simulink model "WaveStar"  (R2018b)
settings: Solver=ode4  StartTime=0  StopTime=141.2  FixedStep=0.001  MaxStep=0.001  RelTol=1e-3  EnableMultiTasking=on
values from neighbouring files (symbols this model uses):
  cc = 10.0    (= 10)    [controller_init.m]
  kc = 0    [controller_init.m]
  L_AB = 0.412    [controller_init.m]
  L_AC = 0.2    [controller_init.m]
  mc = 0    [controller_init.m]
  McSat = inf    [controller_init.m]
  simu = simulationClass()    [wecSimInputFile.m]
  waves = waveClass('irregular')    [wecSimInputFile.m]
  xPcTs = 0.001    [controller_init.m]
undefined symbols (not defined in the file or in its folder): body, constraint, HPfreq, LPfreq, pto, X, Y, Z
libraries: nesl_utility x72, sm_lib x38, WECSim_Lib x7, simulink x2, vrlib x1
(part 2 of 4)

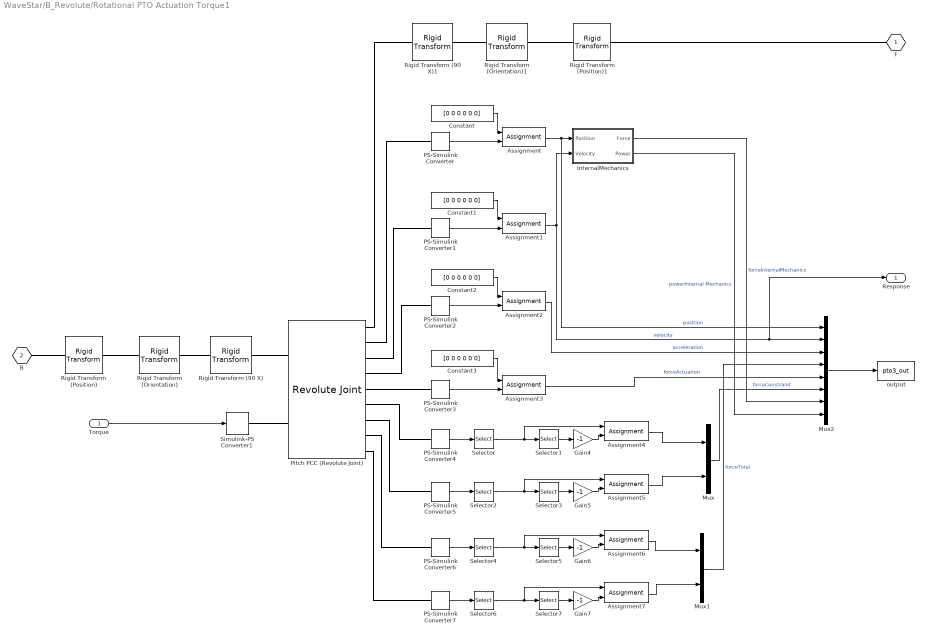
== system WaveStar/B_Revolute/Rotational PTO Actuation Torque1 ==
  Torque : Inport
  "Assignment " : Assignment  IndexOptions=Index vector (dialog)  Indices=5  OutputSizes=1
  Assignment1 : Assignment  IndexOptions=Index vector (dialog)  Indices=5  OutputSizes=1
  Assignment2 : Assignment  IndexOptions=Index vector (dialog)  Indices=5  OutputSizes=1
  Assignment3 : Assignment  IndexOptions=Index vector (dialog)  Indices=5  OutputSizes=1
  Assignment{4..7} (4 alike) : Assignment  DiagnosticForDimensions=Warning  IndexOptions=Index vector (dialog)  Indices=3  OutputSizes=1
  Constant{,1..3} (4 alike) : Constant  Value=[0 0 0 0 0 0]
  Gain{4..7} (4 alike) : Gain  Gain=-1
  InternalMechanics : Subsystem
  Mux : Mux  Inputs=2
  Mux1 : Mux  Inputs=2
  Mux2 : Mux  Inputs=8
  PS-Simulink Converter{,1..7} (8 alike) : nesl_utility/PS-Simulink Converter  PhysicalDomain=network_engine_domain  SubClassName=ps_output  LeftPortType=input  RightPortType=output  PseudoPeriodic=off  Frequencies=[]  Unit=1  AffineConversion=off
  Pitch PCC (Revolute Joint) : sm_lib/Joints/Revolute Joint  SenseConstraintForce=on  SenseConstraintForceX=off  SenseConstraintForceY=off  SenseConstraintForceZ=off  SenseConstraintTorque=on  SenseConstraintTorqueX=off  SenseConstraintTorqueY=off  SenseConstraintTorqueZ=off  SenseTotalForce=on  SenseTotalForceX=off  SenseTotalForceY=off  SenseTotalForceZ=off  SenseTotalTorque=on  SenseTotalTorqueX=off  SenseTotalTorqueY=off  SenseTotalTorqueZ=off  CompositeWrenchDir=BaseOnFollower  CompositeWrenchFrame=BaseFrame  EquilibriumPosition=0  EquilibriumPositionUnits=deg  SpringStiffness=pto.k  SpringStiffnessUnits=N*m/rad  DampingCoefficient=pto.c  DampingCoefficientUnits=N*m/(rad/s)  TorqueActuationMode=InputTorque  MotionActuationMode=ComputedMotion  SensePosition=on  SenseVelocity=on  SenseAcceleration=on  SenseTorqueForce=on  PositionTargetSpecify=off  PositionTargetPriority=High  PositionTargetValue=0  PositionTargetValueUnits=deg  VelocityTargetSpecify=off  VelocityTargetPriority=High  VelocityTargetValue=0  VelocityTargetValueUnits=deg/s
  Rigid Transform (Position) : sm_lib/Frames and Transforms/Rigid Transform  TranslationMethod=Cartesian  TranslationStandardOffset=0  TranslationLengthUnit=m  TranslationStandardAxis=+Z  TranslationCartesianOffset=pto.initDisp.initLinDisp + pto.loc  TranslationROffset=0  TranslationROffsetUnits=m  TranslationZOffset=0  TranslationZOffsetUnits=m  TranslationThetaOffset=0  TranslationThetaOffsetUnits=deg  RotationMethod=None  RotationAngleUnits=rad  RotationStandardAxis=+Y  RotationAngle=0  RotationArbitraryAxis=[0 1 0]  FollAlignAxisA=+X  BaseAlignAxisA=+Y  FollAlignAxisB=+Y  BaseAlignAxisB=+Z  RotationSequenceAxes=FollowerAxes  RotationSequence=XYX  RotationSequenceAngles=[0 0 0]  RotationSequenceAnglesUnits=deg  RotationMatrix=[1 0 0; 0 1 0; 0 0 1]
  Rigid Transform (Position)1 : sm_lib/Frames and Transforms/Rigid Transform  TranslationMethod=Cartesian  TranslationStandardOffset=0  TranslationLengthUnit=m  TranslationStandardAxis=+Z  TranslationCartesianOffset=pto.initDisp.initLinDisp + pto.loc  TranslationROffset=0  TranslationROffsetUnits=m  TranslationZOffset=0  TranslationZOffsetUnits=m  TranslationThetaOffset=0  TranslationThetaOffsetUnits=deg  RotationMethod=None  RotationAngleUnits=rad  RotationStandardAxis=+Y  RotationAngle=0  RotationArbitraryAxis=[0 1 0]  FollAlignAxisA=+X  BaseAlignAxisA=+Y  FollAlignAxisB=+Y  BaseAlignAxisB=+Z  RotationSequenceAxes=FollowerAxes  RotationSequence=XYX  RotationSequenceAngles=[0 0 0]  RotationSequenceAnglesUnits=deg  RotationMatrix=[1 0 0; 0 1 0; 0 0 1]
  Rigid Transform (90 X) : sm_lib/Frames and Transforms/Rigid Transform  TranslationMethod=None  TranslationStandardOffset=0  TranslationLengthUnit=m  TranslationStandardAxis=+Z  TranslationCartesianOffset=0  TranslationROffset=0  TranslationROffsetUnits=m  TranslationZOffset=0  TranslationZOffsetUnits=m  TranslationThetaOffset=0  TranslationThetaOffsetUnits=deg  RotationMethod=StandardAxis  RotationAngleUnits=deg  RotationStandardAxis=+X  RotationAngle=-90  RotationArbitraryAxis=[0 1 0]  FollAlignAxisA=+X  BaseAlignAxisA=+Y  FollAlignAxisB=+Y  BaseAlignAxisB=+Z  RotationSequenceAxes=FollowerAxes  RotationSequence=XYX  RotationSequenceAngles=[0 0 0]  RotationSequenceAnglesUnits=deg  RotationMatrix=[1 0 0; 0 1 0; 0 0 1]
  Rigid Transform (90 X)1 : sm_lib/Frames and Transforms/Rigid Transform  TranslationMethod=None  TranslationStandardOffset=0  TranslationLengthUnit=m  TranslationStandardAxis=+Z  TranslationCartesianOffset=0  TranslationROffset=0  TranslationROffsetUnits=m  TranslationZOffset=0  TranslationZOffsetUnits=m  TranslationThetaOffset=0  TranslationThetaOffsetUnits=deg  RotationMethod=StandardAxis  RotationAngleUnits=deg  RotationStandardAxis=+X  RotationAngle=-90  RotationArbitraryAxis=[0 1 0]  FollAlignAxisA=+X  BaseAlignAxisA=+Y  FollAlignAxisB=+Y  BaseAlignAxisB=+Z  RotationSequenceAxes=FollowerAxes  RotationSequence=XYX  RotationSequenceAngles=[0 0 0]  RotationSequenceAnglesUnits=deg  RotationMatrix=[1 0 0; 0 1 0; 0 0 1]
  Rigid Transform (Orientation) : sm_lib/Frames and Transforms/Rigid Transform  TranslationMethod=None  TranslationStandardOffset=0  TranslationLengthUnit=m  TranslationStandardAxis=+Z  TranslationCartesianOffset=0  TranslationROffset=0  TranslationROffsetUnits=m  TranslationZOffset=0  TranslationZOffsetUnits=m  TranslationThetaOffset=0  TranslationThetaOffsetUnits=deg  RotationMethod=RotationMatrix  RotationAngleUnits=rad  RotationStandardAxis=+Y  RotationAngle=0  RotationArbitraryAxis=[0 1 0]  FollAlignAxisA=+X  BaseAlignAxisA=+Y  FollAlignAxisB=+Y  BaseAlignAxisB=+Z  RotationSequenceAxes=FollowerAxes  RotationSequence=XYX  RotationSequenceAngles=[0 0 0]  RotationSequenceAnglesUnits=deg  RotationMatrix=pto.orientation.rotationMatrix
  Rigid Transform (Orientation)1 : sm_lib/Frames and Transforms/Rigid Transform  TranslationMethod=None  TranslationStandardOffset=0  TranslationLengthUnit=m  TranslationStandardAxis=+Z  TranslationCartesianOffset=0  TranslationROffset=0  TranslationROffsetUnits=m  TranslationZOffset=0  TranslationZOffsetUnits=m  TranslationThetaOffset=0  TranslationThetaOffsetUnits=deg  RotationMethod=RotationMatrix  RotationAngleUnits=rad  RotationStandardAxis=+Y  RotationAngle=0  RotationArbitraryAxis=[0 1 0]  FollAlignAxisA=+X  BaseAlignAxisA=+Y  FollAlignAxisB=+Y  BaseAlignAxisB=+Z  RotationSequenceAxes=FollowerAxes  RotationSequence=XYX  RotationSequenceAngles=[0 0 0]  RotationSequenceAnglesUnits=deg  RotationMatrix=pto.orientation.rotationMatrix
  Selector{,2,4,6} (4 alike) : Selector  InputPortWidth=3  IndexOptions=Index vector (dialog)  Indices=[1 3 2]  OutputSizes=1
  Selector{1,3,5,7} (4 alike) : Selector  InputPortWidth=3  IndexOptions=Index vector (dialog)  Indices=[3]  OutputSizes=1
  Simulink-PS Converter1 : nesl_utility/Simulink-PS Converter  PhysicalDomain=network_engine_domain  SubClassName=ps_input  LeftPortType=input  RightPortType=output  PseudoPeriodic=off  Frequencies=[]  NoiseDistribution=none  NoiseParameters=[]  Unit=1  AffineConversion=off  FilteringAndDerivatives=zero  SimscapeFilterOrder=1  InputFilterTimeConstant=0.001  UdotUserProvided=1
  output : ToWorkspace  VariableName=pto3_out  SaveFormat=Structure With Time  SampleTime=-1
      settings: Decimation=round(simu.dtOut/simu.dt,0)
  F : PMIOPort  Side=Right
  B : PMIOPort  Port=2  Side=Left
  Response : Outport
  wires:
  Torque/1 -> Simulink-PS Converter1/1
  "Assignment "/1 -> Mux2/1, InternalMechanics/1(Position)  "position"
  Assignment1/1 -> Response/1, Mux2/2, InternalMechanics/2(Velocity)  "velocity"
  Assignment2/1 -> Mux2/3  "acceleration"
  Selector2/1 -> Assignment5/1, Selector3/1
  Selector3/1 -> Gain5/1
  Gain5/1 -> Assignment5/2
  Selector/1 -> Assignment4/1, Selector1/1
  Selector1/1 -> Gain4/1
  Gain4/1 -> Assignment4/2
  Assignment5/1 -> Mux/2
  Assignment4/1 -> Mux/1
  Mux/1 -> Mux2/6  "forceConstraint"
  PS-Simulink Converter5/1 -> Selector2/1
  PS-Simulink Converter4/1 -> Selector/1
  Mux2/1 -> output/1
  Mux1/1 -> Mux2/4  "forceTotal"
  Selector6/1 -> Selector7/1, Assignment7/1
  Selector7/1 -> Gain7/1
  Gain7/1 -> Assignment7/2
  Selector4/1 -> Selector5/1, Assignment6/1
  Selector5/1 -> Gain6/1
  Gain6/1 -> Assignment6/2
  PS-Simulink Converter6/1 -> Selector4/1
  PS-Simulink Converter7/1 -> Selector6/1
  Assignment7/1 -> Mux1/2
  Assignment6/1 -> Mux1/1
  Constant/1 -> "Assignment "/1
  PS-Simulink Converter/1 -> "Assignment "/2
  Constant1/1 -> Assignment1/1
  PS-Simulink Converter1/1 -> Assignment1/2
  Constant2/1 -> Assignment2/1
  PS-Simulink Converter2/1 -> Assignment2/2
  Constant3/1 -> Assignment3/1
  PS-Simulink Converter3/1 -> Assignment3/2
  Assignment3/1 -> Mux2/5  "forceActuation"
  InternalMechanics/1(Force) -> Mux2/7  "forceInternalMechanics"
  InternalMechanics/2(Power) -> Mux2/8  "powerInternal Mechanics"
  connections:
  Rigid Transform (Position)1/LConn1 -- F/RConn1
  Rigid Transform (Position)/RConn1 -- Rigid Transform (Orientation)/LConn1
  Rigid Transform (Orientation)/RConn1 -- Rigid Transform (90 X)/LConn1
  Rigid Transform (Orientation)1/RConn1 -- Rigid Transform (90 X)1/LConn1
  Rigid Transform (Position)1/RConn1 -- Rigid Transform (Orientation)1/LConn1
  Rigid Transform (90 X)/RConn1 -- Pitch PCC (Revolute Joint)/LConn1
  Pitch PCC (Revolute Joint)/LConn2 -- Simulink-PS Converter1/RConn1
  Rigid Transform (Position)/LConn1 -- B/RConn1
  PS-Simulink Converter7/LConn1 -- Pitch PCC (Revolute Joint)/RConn9
  PS-Simulink Converter6/LConn1 -- Pitch PCC (Revolute Joint)/RConn8
  PS-Simulink Converter5/LConn1 -- Pitch PCC (Revolute Joint)/RConn7
  PS-Simulink Converter4/LConn1 -- Pitch PCC (Revolute Joint)/RConn6
  Pitch PCC (Revolute Joint)/RConn2 -- PS-Simulink Converter/LConn1
  Pitch PCC (Revolute Joint)/RConn3 -- PS-Simulink Converter1/LConn1
  PS-Simulink Converter2/LConn1 -- Pitch PCC (Revolute Joint)/RConn4
  PS-Simulink Converter3/LConn1 -- Pitch PCC (Revolute Joint)/RConn5
  Rigid Transform (90 X)1/RConn1 -- Pitch PCC (Revolute Joint)/RConn1

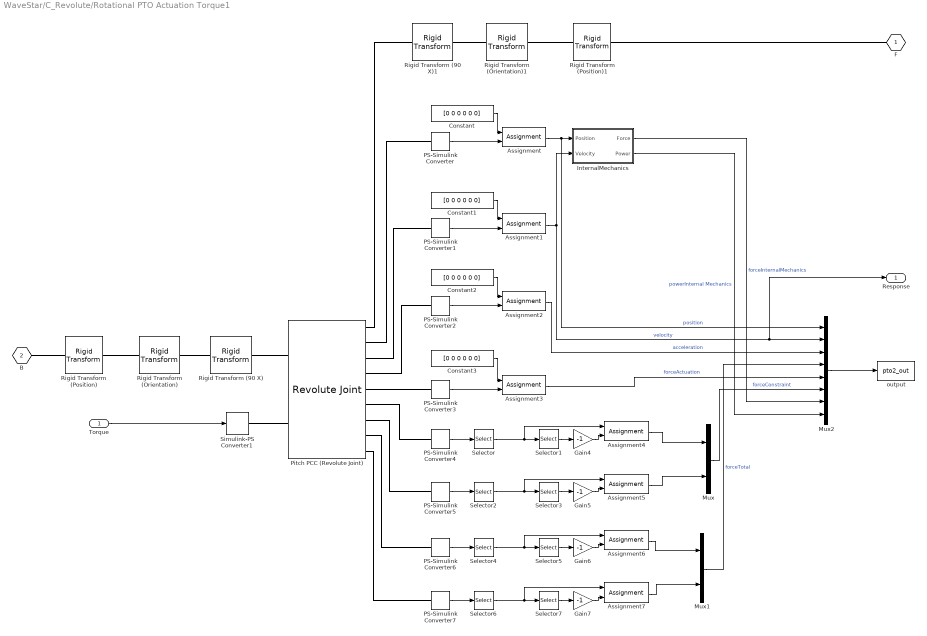
== system WaveStar/C_Revolute/Rotational PTO Actuation Torque1 ==
  Torque : Inport
  "Assignment " : Assignment  IndexOptions=Index vector (dialog)  Indices=5  OutputSizes=1
  Assignment1 : Assignment  IndexOptions=Index vector (dialog)  Indices=5  OutputSizes=1
  Assignment2 : Assignment  IndexOptions=Index vector (dialog)  Indices=5  OutputSizes=1
  Assignment3 : Assignment  IndexOptions=Index vector (dialog)  Indices=5  OutputSizes=1
  Assignment{4..7} (4 alike) : Assignment  DiagnosticForDimensions=Warning  IndexOptions=Index vector (dialog)  Indices=3  OutputSizes=1
  Constant{,1..3} (4 alike) : Constant  Value=[0 0 0 0 0 0]
  Gain{4..7} (4 alike) : Gain  Gain=-1
  InternalMechanics : Subsystem
  Mux : Mux  Inputs=2
  Mux1 : Mux  Inputs=2
  Mux2 : Mux  Inputs=8
  PS-Simulink Converter{,1..7} (8 alike) : nesl_utility/PS-Simulink Converter  PhysicalDomain=network_engine_domain  SubClassName=ps_output  LeftPortType=input  RightPortType=output  PseudoPeriodic=off  Frequencies=[]  Unit=1  AffineConversion=off
  Pitch PCC (Revolute Joint) : sm_lib/Joints/Revolute Joint  SenseConstraintForce=on  SenseConstraintForceX=off  SenseConstraintForceY=off  SenseConstraintForceZ=off  SenseConstraintTorque=on  SenseConstraintTorqueX=off  SenseConstraintTorqueY=off  SenseConstraintTorqueZ=off  SenseTotalForce=on  SenseTotalForceX=off  SenseTotalForceY=off  SenseTotalForceZ=off  SenseTotalTorque=on  SenseTotalTorqueX=off  SenseTotalTorqueY=off  SenseTotalTorqueZ=off  CompositeWrenchDir=BaseOnFollower  CompositeWrenchFrame=BaseFrame  EquilibriumPosition=0  EquilibriumPositionUnits=deg  SpringStiffness=pto.k  SpringStiffnessUnits=N*m/rad  DampingCoefficient=pto.c  DampingCoefficientUnits=N*m/(rad/s)  TorqueActuationMode=InputTorque  MotionActuationMode=ComputedMotion  SensePosition=on  SenseVelocity=on  SenseAcceleration=on  SenseTorqueForce=on  PositionTargetSpecify=off  PositionTargetPriority=High  PositionTargetValue=0  PositionTargetValueUnits=deg  VelocityTargetSpecify=off  VelocityTargetPriority=High  VelocityTargetValue=0  VelocityTargetValueUnits=deg/s
  Rigid Transform (Position) : sm_lib/Frames and Transforms/Rigid Transform  TranslationMethod=Cartesian  TranslationStandardOffset=0  TranslationLengthUnit=m  TranslationStandardAxis=+Z  TranslationCartesianOffset=pto.initDisp.initLinDisp + pto.loc  TranslationROffset=0  TranslationROffsetUnits=m  TranslationZOffset=0  TranslationZOffsetUnits=m  TranslationThetaOffset=0  TranslationThetaOffsetUnits=deg  RotationMethod=None  RotationAngleUnits=rad  RotationStandardAxis=+Y  RotationAngle=0  RotationArbitraryAxis=[0 1 0]  FollAlignAxisA=+X  BaseAlignAxisA=+Y  FollAlignAxisB=+Y  BaseAlignAxisB=+Z  RotationSequenceAxes=FollowerAxes  RotationSequence=XYX  RotationSequenceAngles=[0 0 0]  RotationSequenceAnglesUnits=deg  RotationMatrix=[1 0 0; 0 1 0; 0 0 1]
  Rigid Transform (Position)1 : sm_lib/Frames and Transforms/Rigid Transform  TranslationMethod=Cartesian  TranslationStandardOffset=0  TranslationLengthUnit=m  TranslationStandardAxis=+Z  TranslationCartesianOffset=pto.initDisp.initLinDisp + pto.loc  TranslationROffset=0  TranslationROffsetUnits=m  TranslationZOffset=0  TranslationZOffsetUnits=m  TranslationThetaOffset=0  TranslationThetaOffsetUnits=deg  RotationMethod=None  RotationAngleUnits=rad  RotationStandardAxis=+Y  RotationAngle=0  RotationArbitraryAxis=[0 1 0]  FollAlignAxisA=+X  BaseAlignAxisA=+Y  FollAlignAxisB=+Y  BaseAlignAxisB=+Z  RotationSequenceAxes=FollowerAxes  RotationSequence=XYX  RotationSequenceAngles=[0 0 0]  RotationSequenceAnglesUnits=deg  RotationMatrix=[1 0 0; 0 1 0; 0 0 1]
  Rigid Transform (90 X) : sm_lib/Frames and Transforms/Rigid Transform  TranslationMethod=None  TranslationStandardOffset=0  TranslationLengthUnit=m  TranslationStandardAxis=+Z  TranslationCartesianOffset=0  TranslationROffset=0  TranslationROffsetUnits=m  TranslationZOffset=0  TranslationZOffsetUnits=m  TranslationThetaOffset=0  TranslationThetaOffsetUnits=deg  RotationMethod=StandardAxis  RotationAngleUnits=deg  RotationStandardAxis=+X  RotationAngle=-90  RotationArbitraryAxis=[0 1 0]  FollAlignAxisA=+X  BaseAlignAxisA=+Y  FollAlignAxisB=+Y  BaseAlignAxisB=+Z  RotationSequenceAxes=FollowerAxes  RotationSequence=XYX  RotationSequenceAngles=[0 0 0]  RotationSequenceAnglesUnits=deg  RotationMatrix=[1 0 0; 0 1 0; 0 0 1]
  Rigid Transform (90 X)1 : sm_lib/Frames and Transforms/Rigid Transform  TranslationMethod=None  TranslationStandardOffset=0  TranslationLengthUnit=m  TranslationStandardAxis=+Z  TranslationCartesianOffset=0  TranslationROffset=0  TranslationROffsetUnits=m  TranslationZOffset=0  TranslationZOffsetUnits=m  TranslationThetaOffset=0  TranslationThetaOffsetUnits=deg  RotationMethod=StandardAxis  RotationAngleUnits=deg  RotationStandardAxis=+X  RotationAngle=-90  RotationArbitraryAxis=[0 1 0]  FollAlignAxisA=+X  BaseAlignAxisA=+Y  FollAlignAxisB=+Y  BaseAlignAxisB=+Z  RotationSequenceAxes=FollowerAxes  RotationSequence=XYX  RotationSequenceAngles=[0 0 0]  RotationSequenceAnglesUnits=deg  RotationMatrix=[1 0 0; 0 1 0; 0 0 1]
  Rigid Transform (Orientation) : sm_lib/Frames and Transforms/Rigid Transform  TranslationMethod=None  TranslationStandardOffset=0  TranslationLengthUnit=m  TranslationStandardAxis=+Z  TranslationCartesianOffset=0  TranslationROffset=0  TranslationROffsetUnits=m  TranslationZOffset=0  TranslationZOffsetUnits=m  TranslationThetaOffset=0  TranslationThetaOffsetUnits=deg  RotationMethod=RotationMatrix  RotationAngleUnits=rad  RotationStandardAxis=+Y  RotationAngle=0  RotationArbitraryAxis=[0 1 0]  FollAlignAxisA=+X  BaseAlignAxisA=+Y  FollAlignAxisB=+Y  BaseAlignAxisB=+Z  RotationSequenceAxes=FollowerAxes  RotationSequence=XYX  RotationSequenceAngles=[0 0 0]  RotationSequenceAnglesUnits=deg  RotationMatrix=pto.orientation.rotationMatrix
  Rigid Transform (Orientation)1 : sm_lib/Frames and Transforms/Rigid Transform  TranslationMethod=None  TranslationStandardOffset=0  TranslationLengthUnit=m  TranslationStandardAxis=+Z  TranslationCartesianOffset=0  TranslationROffset=0  TranslationROffsetUnits=m  TranslationZOffset=0  TranslationZOffsetUnits=m  TranslationThetaOffset=0  TranslationThetaOffsetUnits=deg  RotationMethod=RotationMatrix  RotationAngleUnits=rad  RotationStandardAxis=+Y  RotationAngle=0  RotationArbitraryAxis=[0 1 0]  FollAlignAxisA=+X  BaseAlignAxisA=+Y  FollAlignAxisB=+Y  BaseAlignAxisB=+Z  RotationSequenceAxes=FollowerAxes  RotationSequence=XYX  RotationSequenceAngles=[0 0 0]  RotationSequenceAnglesUnits=deg  RotationMatrix=pto.orientation.rotationMatrix
  Selector{,2,4,6} (4 alike) : Selector  InputPortWidth=3  IndexOptions=Index vector (dialog)  Indices=[1 3 2]  OutputSizes=1
  Selector{1,3,5,7} (4 alike) : Selector  InputPortWidth=3  IndexOptions=Index vector (dialog)  Indices=[3]  OutputSizes=1
  Simulink-PS Converter1 : nesl_utility/Simulink-PS Converter  PhysicalDomain=network_engine_domain  SubClassName=ps_input  LeftPortType=input  RightPortType=output  PseudoPeriodic=off  Frequencies=[]  NoiseDistribution=none  NoiseParameters=[]  Unit=1  AffineConversion=off  FilteringAndDerivatives=zero  SimscapeFilterOrder=1  InputFilterTimeConstant=0.001  UdotUserProvided=1
  output : ToWorkspace  VariableName=pto2_out  SaveFormat=Structure With Time  SampleTime=-1
      settings: Decimation=round(simu.dtOut/simu.dt,0)
  F : PMIOPort  Side=Right
  B : PMIOPort  Port=2  Side=Left
  Response : Outport
  wires:
  Torque/1 -> Simulink-PS Converter1/1
  "Assignment "/1 -> Mux2/1, InternalMechanics/1(Position)  "position"
  Assignment1/1 -> Response/1, Mux2/2, InternalMechanics/2(Velocity)  "velocity"
  Assignment2/1 -> Mux2/3  "acceleration"
  Selector2/1 -> Assignment5/1, Selector3/1
  Selector3/1 -> Gain5/1
  Gain5/1 -> Assignment5/2
  Selector/1 -> Assignment4/1, Selector1/1
  Selector1/1 -> Gain4/1
  Gain4/1 -> Assignment4/2
  Assignment5/1 -> Mux/2
  Assignment4/1 -> Mux/1
  Mux/1 -> Mux2/6  "forceConstraint"
  PS-Simulink Converter5/1 -> Selector2/1
  PS-Simulink Converter4/1 -> Selector/1
  Mux2/1 -> output/1
  Mux1/1 -> Mux2/4  "forceTotal"
  Selector6/1 -> Selector7/1, Assignment7/1
  Selector7/1 -> Gain7/1
  Gain7/1 -> Assignment7/2
  Selector4/1 -> Selector5/1, Assignment6/1
  Selector5/1 -> Gain6/1
  Gain6/1 -> Assignment6/2
  PS-Simulink Converter6/1 -> Selector4/1
  PS-Simulink Converter7/1 -> Selector6/1
  Assignment7/1 -> Mux1/2
  Assignment6/1 -> Mux1/1
  Constant/1 -> "Assignment "/1
  PS-Simulink Converter/1 -> "Assignment "/2
  Constant1/1 -> Assignment1/1
  PS-Simulink Converter1/1 -> Assignment1/2
  Constant2/1 -> Assignment2/1
  PS-Simulink Converter2/1 -> Assignment2/2
  Constant3/1 -> Assignment3/1
  PS-Simulink Converter3/1 -> Assignment3/2
  Assignment3/1 -> Mux2/5  "forceActuation"
  InternalMechanics/1(Force) -> Mux2/7  "forceInternalMechanics"
  InternalMechanics/2(Power) -> Mux2/8  "powerInternal Mechanics"
  connections:
  Rigid Transform (Position)1/LConn1 -- F/RConn1
  Rigid Transform (Position)/RConn1 -- Rigid Transform (Orientation)/LConn1
  Rigid Transform (Orientation)/RConn1 -- Rigid Transform (90 X)/LConn1
  Rigid Transform (Orientation)1/RConn1 -- Rigid Transform (90 X)1/LConn1
  Rigid Transform (Position)1/RConn1 -- Rigid Transform (Orientation)1/LConn1
  Rigid Transform (90 X)/RConn1 -- Pitch PCC (Revolute Joint)/LConn1
  Pitch PCC (Revolute Joint)/LConn2 -- Simulink-PS Converter1/RConn1
  Rigid Transform (Position)/LConn1 -- B/RConn1
  PS-Simulink Converter7/LConn1 -- Pitch PCC (Revolute Joint)/RConn9
  PS-Simulink Converter6/LConn1 -- Pitch PCC (Revolute Joint)/RConn8
  PS-Simulink Converter5/LConn1 -- Pitch PCC (Revolute Joint)/RConn7
  PS-Simulink Converter4/LConn1 -- Pitch PCC (Revolute Joint)/RConn6
  Pitch PCC (Revolute Joint)/RConn2 -- PS-Simulink Converter/LConn1
  Pitch PCC (Revolute Joint)/RConn3 -- PS-Simulink Converter1/LConn1
  PS-Simulink Converter2/LConn1 -- Pitch PCC (Revolute Joint)/RConn4
  PS-Simulink Converter3/LConn1 -- Pitch PCC (Revolute Joint)/RConn5
  Rigid Transform (90 X)1/RConn1 -- Pitch PCC (Revolute Joint)/RConn1

== system WaveStar/Controller/Linear ==
  wave_gauge_1 : Inport
  wave_gauge_2 : Inport  Port=2
  wave_gauge_3 : Inport  Port=3
  float_accel : Inport  Port=4
  motor_force : Inport  Port=5
  "motor_pos " : Inport  Port=6
  WECCCOMP Controller : Subsystem
  cmd_force : Outport
  wires:
  WECCCOMP Controller/1(cmd_force) -> cmd_force/1
  float_accel/1 -> WECCCOMP Controller/1(float_accel_rot)
  motor_force/1 -> WECCCOMP Controller/2(motor_force)
  "motor_pos "/1 -> WECCCOMP Controller/3("motor_pos ")
  wave_gauge_1/1 -> WECCCOMP Controller/4(wave_gauge_1)
  wave_gauge_2/1 -> WECCCOMP Controller/5(wave_gauge_2)
  wave_gauge_3/1 -> WECCCOMP Controller/6(wave_gauge_3)

== system WaveStar/Controller/Rotary ==
  wave_gauge_1 : Inport
  wave_gauge_2 : Inport  Port=2
  wave_gauge_3 : Inport  Port=3
  float_accel : Inport  Port=4
  motor_force : Inport  Port=5
  "motor_pos " : Inport  Port=6
  MATLAB Function : MATLAB Function  TreatAsAtomicUnit=on
  Ramp : simulink/Sources/Ramp  slope=1  start=0  InitialOutput=0
  Rate Transition1 : RateTransition  OutPortSampleTime=simu.dt
  WECCCOMP Controller : Subsystem
  lin2rot conversion : Subsystem
  rot2lin conversion : Subsystem
  cmd_force : Outport
  wires:
  float_accel/1 -> lin2rot conversion/1(float_accel)
  motor_force/1 -> lin2rot conversion/2(motor_force)
  "motor_pos "/1 -> lin2rot conversion/3("motor_pos ")
  rot2lin conversion/1(cmd_force) -> cmd_force/1
  WECCCOMP Controller/1(cmd_torque_rot) -> rot2lin conversion/1(cmd_torque_rot)
  lin2rot conversion/2(motor_torque_rot) -> WECCCOMP Controller/2(motor_torque_rot)
  lin2rot conversion/1("float_accel_rot ") -> MATLAB Function/4(float_accel)
  lin2rot conversion/3(motor_pos_rot) -> MATLAB Function/6(pos)
  wave_gauge_1/1 -> MATLAB Function/1(ws1)
  lin2rot conversion/4(moment_arm) -> rot2lin conversion/2(moment_arm)
  wave_gauge_2/1 -> MATLAB Function/2(ws2)
  wave_gauge_3/1 -> MATLAB Function/3(ws3)
  MATLAB Function/1(WS1) -> WECCCOMP Controller/4(wave_gauge_1)
  MATLAB Function/2(WS2) -> WECCCOMP Controller/5(wave_gauge_2)
  MATLAB Function/3(WS3) -> WECCCOMP Controller/6(wave_gauge_3)
  MATLAB Function/4(ACC) -> WECCCOMP Controller/1(float_accel_rot)
  MATLAB Function/5(POS) -> WECCCOMP Controller/3("motor_pos_rot ")
  Ramp/1 -> Rate Transition1/1
  Rate Transition1/1 -> MATLAB Function/5(time)

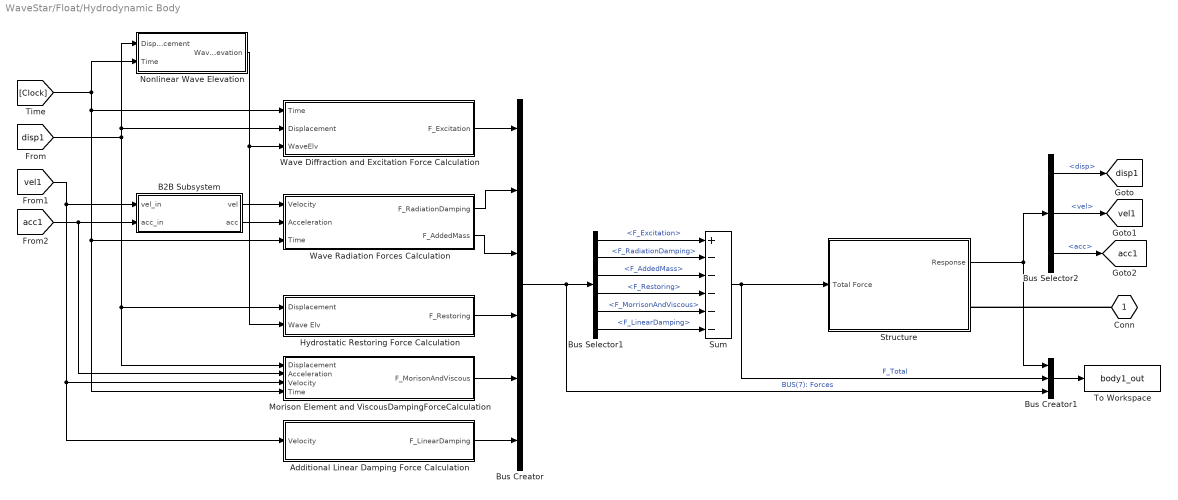
== system WaveStar/Float/Hydrodynamic Body ==
  Additional Linear Damping Force Calculation : Subsystem
  B2B Subsystem : Subsystem  Variant=on
  Bus Creator : BusCreator  Inputs=6
  Bus Creator1 : BusCreator  Inputs=3
  Bus Selector1 : BusSelector  OutputSignals=F_Excitation,F_RadiationDamping,F_AddedMass,F_Restoring,F_MorrisonAndViscous,F_LinearDamping
  Bus Selector2 : BusSelector  OutputSignals=disp,vel,acc
  Hydrostatic Restoring Force Calculation : Subsystem
  Morison Element and ViscousDampingForceCalculation : Subsystem
  Nonlinear Wave Elevation : Subsystem  TreatAsAtomicUnit=on  SystemSampleTime=simu.dtNL
  Structure : Subsystem
  Sum : Sum  Inputs=+-----
  To Workspace : ToWorkspace  VariableName=body1_out  SaveFormat=Structure With Time  SampleTime=-1
      settings: Decimation=round(simu.dtOut/simu.dt,0)
  Wave Diffraction and Excitation Force Calculation : Subsystem
  Wave Radiation Forces Calculation : Subsystem
  Conn : PMIOPort  Side=Right
  tag scope: acc1=global, disp1=global, vel1=global
  wires:
  Additional Linear Damping Force Calculation/1(F_LinearDamping) -> Bus Creator/6
  Bus Creator/1 -> Bus Selector1/1, Bus Creator1/3  "BUS(7): Forces"
  Bus Selector2/1 -> [disp1]  "<disp>"
  Bus Selector2/3 -> [acc1]  "<acc>"
  Bus Selector2/2 -> [vel1]  "<vel>"
  Structure/1(Response) -> Bus Creator1/1, Bus Selector2/1
  Sum/1 -> Bus Creator1/2, Structure/1(Total Force)  "F_Total"
  Bus Creator1/1 -> To Workspace/1
  Bus Selector1/4 -> Sum/4  "<F_Restoring>"
  Bus Selector1/3 -> Sum/3  "<F_AddedMass>"
  Bus Selector1/5 -> Sum/5  "<F_MorrisonAndViscous>"
  Bus Selector1/2 -> Sum/2  "<F_RadiationDamping>"
  Bus Selector1/1 -> Sum/1  "<F_Excitation>"
  Bus Selector1/6 -> Sum/6  "<F_LinearDamping>"
  [acc1] -> B2B Subsystem/2(acc_in), Morison Element and ViscousDampingForceCalculation/2(Acceleration)
  [vel1] -> Morison Element and ViscousDampingForceCalculation/3(Velocity), Additional Linear Damping Force Calculation/1(Velocity), B2B Subsystem/1(vel_in)
  B2B Subsystem/2(acc) -> Wave Radiation Forces Calculation/2(Acceleration)
  B2B Subsystem/1(vel) -> Wave Radiation Forces Calculation/1(Velocity)
  [disp1] -> Hydrostatic Restoring Force Calculation/1(Displacement), Morison Element and ViscousDampingForceCalculation/1(Displacement), Nonlinear Wave Elevation/1(Displacement), Wave Diffraction and Excitation Force Calculation/2(Displacement)
  Nonlinear Wave Elevation/1(Wave Elevation) -> Wave Diffraction and Excitation Force Calculation/3(WaveElv), Hydrostatic Restoring Force Calculation/2(Wave Elv)
  Hydrostatic Restoring Force Calculation/1(F_Restoring) -> Bus Creator/4
  Wave Radiation Forces Calculation/1(F_RadiationDamping) -> Bus Creator/2
  Wave Diffraction and Excitation Force Calculation/1(F_Excitation) -> Bus Creator/1
  Wave Radiation Forces Calculation/2(F_AddedMass) -> Bus Creator/3
  [Clock] -> Nonlinear Wave Elevation/2(Time), Wave Diffraction and Excitation Force Calculation/1(Time), Morison Element and ViscousDampingForceCalculation/4(Time), Wave Radiation Forces Calculation/3(Time)
  Morison Element and ViscousDampingForceCalculation/1(F_MorisonAndViscous) -> Bus Creator/5
  connections:
  Conn/RConn1 -- Structure/RConn1

== system WaveStar/Float/Non-Hydro Body ==
  Bus Creator : BusCreator  Inputs=6
  Bus Creator1 : BusCreator  Inputs=3
  Bus Selector1 : BusSelector  OutputSignals=F_Excitation,F_RadiationDamping,F_AddedMass,F_Restoring,F_MorrisonAndViscous,F_LinearDamping
  Constant{,1..3,5} (5 alike) : Constant  Value=[0 0 0 0 0 0]
  Structure : Subsystem
  Sum : Sum  Inputs=+-----
  To Workspace : ToWorkspace  VariableName=body1_out  SaveFormat=Structure With Time  SampleTime=-1
      settings: Decimation=round(simu.dtOut/simu.dt,0)
  Weight and Buoyancy : Subsystem
  Conn : PMIOPort  Side=Right
  wires:
  Bus Creator/1 -> Bus Creator1/3, Bus Selector1/1  "BUS(7): Forces"
  Structure/1(Response) -> Bus Creator1/1
  Sum/1 -> Bus Creator1/2, Structure/1(Total Force)  "F_Total"
  Bus Creator1/1 -> To Workspace/1
  Bus Selector1/4 -> Sum/4  "<F_Restoring>"
  Bus Selector1/3 -> Sum/3  "<F_AddedMass>"
  Bus Selector1/5 -> Sum/5  "<F_MorrisonAndViscous>"
  Bus Selector1/2 -> Sum/2  "<F_RadiationDamping>"
  Bus Selector1/1 -> Sum/1  "<F_Excitation>"
  Bus Selector1/6 -> Sum/6  "<F_LinearDamping>"
  Constant5/1 -> Bus Creator/6  "F_LinearDamping"
  Constant3/1 -> Bus Creator/5  "F_MorrisonAndViscous"
  Constant2/1 -> Bus Creator/3  "F_AddedMass"
  Constant1/1 -> Bus Creator/2  "F_RadiationDamping"
  Constant/1 -> Bus Creator/1  "F_Excitation"
  Weight and Buoyancy/1(Out1) -> Bus Creator/4  "F_Restoring"
  connections:
  Conn/RConn1 -- Structure/RConn1

== system WaveStar/Linear Motor/InternalMechanics ==
  note: Calculate PTO force and power.
      |
      | F_pto  = k*x + c*v,
      | where F_pto is the force the PTO applies to the body (at the PTO location), x and v are the joint position and velocity.
      |
      | The power extracted is
      | P = c * v^2
  Position : Inport
  Velocity : Inport  Port=2
  Add : Sum  Inputs=--
  Math Function : Math  Operator=square  SaturateOnIntegerOverflow=on
  PCC Damping Coefficient : Constant  Value=pto.c
  PCC Stiffness Coefficient : Constant  Value=pto.k
  Product : Product  Inputs=**
  Product1 : Product  Inputs=**
  Product2 : Product  Inputs=**
  Force : Outport
  Power : Outport  Port=2
  wires:
  PCC Damping Coefficient/1 -> Product2/1, Product1/1
  Product2/1 -> Power/1
  Velocity/1 -> Math Function/1, Product1/2
  PCC Stiffness Coefficient/1 -> Product/2
  Position/1 -> Product/1
  Add/1 -> Force/1
  Math Function/1 -> Product2/2
  Product/1 -> Add/1
  Product1/1 -> Add/2

== system WaveStar/A_Revolute/Rotational PTO Actuation Torque1/InternalMechanics ==
  note: Calculate PTO force and power.
      |
      | F_pto  = k*x + c*v,
      | where F_pto is the force the PTO applies to the body (at the PTO location), x and v are the joint position and velocity.
      |
      | The power extracted is
      | P_pto = F_pto * v
  Position : Inport
  Velocity : Inport  Port=2
  Add : Sum  Inputs=--
  PCC Damping Coefficient : Constant  Value=pto.c
  PCC Stiffness Coefficient : Constant  Value=pto.k
  Product : Product  Inputs=**
  Product1 : Product  Inputs=**
  Product2 : Product  Inputs=**
  Force : Outport
  Power : Outport  Port=2
  wires:
  PCC Damping Coefficient/1 -> Product1/1
  Product2/1 -> Power/1
  PCC Stiffness Coefficient/1 -> Product/2
  Position/1 -> Product/1
  Add/1 -> Force/1, Product2/1
  Velocity/1 -> Product1/2, Product2/2
  Product/1 -> Add/1
  Product1/1 -> Add/2

== system WaveStar/B_Revolute/Rotational PTO Actuation Torque1/InternalMechanics ==
  note: Calculate PTO force and power.
      |
      | F_pto  = k*x + c*v,
      | where F_pto is the force the PTO applies to the body (at the PTO location), x and v are the joint position and velocity.
      |
      | The power extracted is
      | P_pto = F_pto * v
  Position : Inport
  Velocity : Inport  Port=2
  Add : Sum  Inputs=--
  PCC Damping Coefficient : Constant  Value=pto.c
  PCC Stiffness Coefficient : Constant  Value=pto.k
  Product : Product  Inputs=**
  Product1 : Product  Inputs=**
  Product2 : Product  Inputs=**
  Force : Outport
  Power : Outport  Port=2
  wires:
  PCC Damping Coefficient/1 -> Product1/1
  Product2/1 -> Power/1
  PCC Stiffness Coefficient/1 -> Product/2
  Position/1 -> Product/1
  Add/1 -> Force/1, Product2/1
  Velocity/1 -> Product1/2, Product2/2
  Product/1 -> Add/1
  Product1/1 -> Add/2

== system WaveStar/C_Revolute/Rotational PTO Actuation Torque1/InternalMechanics ==
  note: Calculate PTO force and power.
      |
      | F_pto  = k*x + c*v,
      | where F_pto is the force the PTO applies to the body (at the PTO location), x and v are the joint position and velocity.
      |
      | The power extracted is
      | P_pto = F_pto * v
  Position : Inport
  Velocity : Inport  Port=2
  Add : Sum  Inputs=--
  PCC Damping Coefficient : Constant  Value=pto.c
  PCC Stiffness Coefficient : Constant  Value=pto.k
  Product : Product  Inputs=**
  Product1 : Product  Inputs=**
  Product2 : Product  Inputs=**
  Force : Outport
  Power : Outport  Port=2
  wires:
  PCC Damping Coefficient/1 -> Product1/1
  Product2/1 -> Power/1
  PCC Stiffness Coefficient/1 -> Product/2
  Position/1 -> Product/1
  Add/1 -> Force/1, Product2/1
  Velocity/1 -> Product1/2, Product2/2
  Product/1 -> Add/1
  Product1/1 -> Add/2

== system WaveStar/Controller/Linear/WECCCOMP Controller ==
  float_accel_rot : Inport
  motor_force : Inport  Port=2
  "motor_pos " : Inport  Port=3
  wave_gauge_1 : Inport  Port=4
  wave_gauge_2 : Inport  Port=5
  wave_gauge_3 : Inport  Port=6
  Constant : Constant  Value=0
  Terminator{,1..5} (6 alike) : Terminator
  lin2rot conversion : Subsystem
  rot2lin conversion : Subsystem
  cmd_force : Outport
  wires:
  lin2rot conversion/2(moment_arm) -> rot2lin conversion/2(moment_arm)
  wave_gauge_1/1 -> Terminator/1
  "motor_pos "/1 -> lin2rot conversion/2("motor_pos ")
  motor_force/1 -> Terminator2/1
  float_accel_rot/1 -> lin2rot conversion/1(float_accel_rot)
  rot2lin conversion/1(cmd_force) -> cmd_force/1
  Constant/1 -> rot2lin conversion/1(cmd_force_ref)
  lin2rot conversion/1("float_accel ") -> Terminator1/1
  lin2rot conversion/3(motor_vel) -> Terminator4/1
  wave_gauge_2/1 -> Terminator3/1
  wave_gauge_3/1 -> Terminator5/1

== system WaveStar/Controller/Rotary/WECCCOMP Controller ==
  float_accel_rot : Inport
  motor_torque_rot : Inport  Port=2
  "motor_pos_rot " : Inport  Port=3
  wave_gauge_1 : Inport  Port=4
  wave_gauge_2 : Inport  Port=5
  wave_gauge_3 : Inport  Port=6
  Differentiator with break frequency : DiscreteTransferFcn  Numerator=[1 -1]*2*2*pi*HPfreq.vel  Denominator=[(2+2*pi*HPfreq.vel*xPcTs) (2*pi*HPfreq.vel*xPcTs-2)]
  First order LP filter : DiscreteTransferFcn  Numerator=[1 1]*xPcTs*2*pi*LPfreq.vel  Denominator=[(2+xPcTs*2*pi*LPfreq.vel) (xPcTs*2*pi*LPfreq.vel-2)]
  Sum1 : Sum  Inputs=+++
  cc : Gain  Gain=cc
  kc : Gain  Gain=kc
  mc : Gain  Gain=mc
  motor torque terminator : Terminator
  wave gauge 1 terminator : Terminator
  wave gauge 2 terminator : Terminator
  wave gauge 3 terminator : Terminator
  cmd_torque_rot : Outport
  wires:
  cc/1 -> Sum1/2
  kc/1 -> Sum1/3
  "motor_pos_rot "/1 -> Differentiator with break frequency/1, kc/1
  float_accel_rot/1 -> mc/1
  mc/1 -> Sum1/1
  motor_torque_rot/1 -> motor torque terminator/1
  wave_gauge_1/1 -> wave gauge 1 terminator/1
  Differentiator with break frequency/1 -> First order LP filter/1
  First order LP filter/1 -> cc/1
  Sum1/1 -> cmd_torque_rot/1  "Mc"
  wave_gauge_2/1 -> wave gauge 2 terminator/1
  wave_gauge_3/1 -> wave gauge 3 terminator/1

== system WaveStar/Controller/Rotary/lin2rot conversion ==
  float_accel : Inport
  motor_force : Inport  Port=2
  "motor_pos " : Inport  Port=3
  Axial Motor Force : Selector  InputPortWidth=6  IndexOptions=Index vector (dialog)  Indices=[3]  OutputSizes=1
  Axial Position : Selector  InputPortWidth=6  IndexOptions=Index vector (dialog)  Indices=[3]  OutputSizes=1
  Divide => K (m)2 : Product  Inputs=**
  Linear2Angular Conversion : Subsystem
  "float_accel_rot " : Outport
  motor_torque_rot : Outport  Port=2
  motor_pos_rot : Outport  Port=3
  moment_arm : Outport  Port=4
  wires:
  "motor_pos "/1 -> Axial Position/1
  Linear2Angular Conversion/2(moment_arm) -> Divide => K (m)2/1, moment_arm/1
  Axial Position/1 -> Linear2Angular Conversion/1(x_cyl)
  Linear2Angular Conversion/1(Theta) -> motor_pos_rot/1
  float_accel/1 -> "float_accel_rot "/1  "Angular Acceleration"
  motor_force/1 -> Axial Motor Force/1
  Axial Motor Force/1 -> Divide => K (m)2/2
  Divide => K (m)2/1 -> motor_torque_rot/1

== system WaveStar/Controller/Rotary/rot2lin conversion ==
  cmd_torque_rot : Inport
  moment_arm : Inport  Port=2
  Cmd torque to measured torque dynamics : DiscreteTransferFcn  Numerator="[0.96294775   -1.92342278    0.96053421]"  Denominator="[1.00000000   -1.99777700    0.99783206]"
  "Divide " : Product  Inputs=*/
  Gain : Gain  Gain=-1
  Saturation : Saturate  UpperLimit=McSat  LowerLimit=-McSat
  cmd_force : Outport
  wires:
  "Divide "/1 -> cmd_force/1
  moment_arm/1 -> "Divide "/2
  Saturation/1 -> Gain/1  "Mc_sat"
  Gain/1 -> "Divide "/1
  cmd_torque_rot/1 -> Cmd torque to measured torque dynamics/1
  Cmd torque to measured torque dynamics/1 -> Saturation/1

== system WaveStar/Float/Hydrodynamic Body/Additional Linear Damping Force Calculation ==
  Velocity : Inport
  Additional Linear Damping Matrix (diagonal) : Constant  Value=body.hydroForce.linearDamping
  Product1 : Product
  F_LinearDamping : Outport
  wires:
  Velocity/1 -> Product1/2  "v"
  Product1/1 -> F_LinearDamping/1  "F_LinearDamping"
  Additional Linear Damping Matrix (diagonal)/1 -> Product1/1  "C"

== system WaveStar/Float/Hydrodynamic Body/B2B Subsystem ==
  note: 1) Add Subsystem or Model blocks as valid variant choices.
      | 2) You cannot connect blocks at this level. At simulation, connectivity is automatically
      | determined, based on the active variant and port name matching.
  vel_in : Inport
  acc_in : Inport  Port=2
  B2B : Subsystem  VariantControl=sv_B2B
  noB2B : Subsystem  VariantControl=sv_noB2B
  vel : Outport
  acc : Outport  Port=2

== system WaveStar/Float/Hydrodynamic Body/Hydrostatic Restoring Force Calculation ==
  Displacement : Inport
  Wave Elv : Inport  Port=2
  Add : Sum  Inputs=+-
  Center of Gravity : Constant  Value=body.cg
  Constant : Constant  Value=zeros(1,body.dof-3)
  Linear and Nonlinear Restoring Force Variant Subsystem : Subsystem  Variant=on
  Mux : Mux  Inputs=2
  F_Restoring : Outport
  wires:
  Add/1 -> Linear and Nonlinear Restoring Force Variant Subsystem/1(In1)  "x_cg"
  Wave Elv/1 -> Linear and Nonlinear Restoring Force Variant Subsystem/2(In2)
  Constant/1 -> Mux/2
  Center of Gravity/1 -> Mux/1  "cg"
  Mux/1 -> Add/2
  Linear and Nonlinear Restoring Force Variant Subsystem/1(Out1) -> F_Restoring/1  "F_Restoring"
  Displacement/1 -> Add/1  "x"

== system WaveStar/Float/Hydrodynamic Body/Morison Element and ViscousDampingForceCalculation ==
  Displacement : Inport
  Acceleration : Inport  Port=2
  Velocity : Inport  Port=3
  Time : Inport  Port=4
  Abs1 : Abs
  Morison Element Variant Subsystem : Subsystem  Variant=on
  Product : Product
  Product1 : Product  Multiplication=Matrix(*)
  Transport Delay : TransportDelay  DelayTime=10e-8
  "VisSum " : Sum  Inputs=+-
  "Viscous Damping Matrix (diagonal) " : Constant  Value=body.hydroForce.visDrag
  F_MorisonAndViscous : Outport
  wires:
  Morison Element Variant Subsystem/1(morison_force) -> "VisSum "/2
  Velocity/1 -> Abs1/1, Morison Element Variant Subsystem/2(velocity), Product/1
  Transport Delay/1 -> Morison Element Variant Subsystem/3(acceleration)
  Displacement/1 -> Morison Element Variant Subsystem/1(displacement)
  Time/1 -> Morison Element Variant Subsystem/4(time)
  Product/1 -> Product1/2  "v * |v|"
  "Viscous Damping Matrix (diagonal) "/1 -> Product1/1  "0.5 * cd * rho *A"
  Product1/1 -> "VisSum "/1
  Abs1/1 -> Product/2
  Acceleration/1 -> Transport Delay/1
  "VisSum "/1 -> F_MorisonAndViscous/1  "F_MorrisonAndViscous"

== system WaveStar/Float/Hydrodynamic Body/Nonlinear Wave Elevation ==
  Displacement : Inport
  Time : Inport  Port=2
  Add : Sum  Inputs=+-
  Center of Gravity : Constant  Value=body.cg
  Constant : Constant  Value=zeros(1,body.dof-3)
  Linear or Instantaneous Free Surface : Subsystem  Variant=on
  Mux : Mux  Inputs=2
  Wave Elevation : Outport
  wires:
  Time/1 -> Linear or Instantaneous Free Surface/2(In2)
  Constant/1 -> Mux/2
  Center of Gravity/1 -> Mux/1  "cg"
  Mux/1 -> Add/2
  Add/1 -> Linear or Instantaneous Free Surface/1(In1)  "x_cg"
  Linear or Instantaneous Free Surface/1(Out1) -> Wave Elevation/1
  Displacement/1 -> Add/1  "x"

== system WaveStar/Float/Hydrodynamic Body/Structure ==
  Total Force : Inport
  Body Properties : sm_lib/Body Elements/Solid  InertiaType=Custom  Mass=body.mass  MassUnits=kg  CenterOfMass=[0 0 0]  CenterOfMassUnits=m  MomentsOfInertia=body.momOfInertia  MomentsOfInertiaUnits=kg*m^2  ProductsOfInertia=[0 0 0]  ProductsOfInertiaUnits=kg*m^2  BasedOnType=Density  Density=1000  DensityUnits=kg/(m^3)  DoExposeReferenceFrame=on  SerializedFrames=<Frames/>  GraphicType=FromGeometry  MarkerShape=Sphere  MarkerSize=10  MarkerSizeUnits=m  GraphicVisPropType=SimpleVisualProperties  GraphicDiffuseColor=body.viz.color  GraphicSpecularColor=[0.5 0.5 0.5 1.0]  GraphicAmbientColor=[0.15 0.15 0.15 1.0]  GraphicEmissiveColor=[0.0 0.0 0.0 1.0]  GraphicShininess=75  GraphicOpacity=body.viz.opacity  GeometryShape=FromFile  RectangleSize=[1 1]  RectangleSizeUnits=m  BrickDimensions=[1 1 1]  BrickDimensionUnits=m  CylinderRadius=1  CylinderRadiusUnits=m  CylinderLength=1  CylinderLengthUnits=m  SphereRadius=1  SphereRadiusUnits=m  EllipsoidRadii=[1 1 1]  EllipsoidRadiiUnits=m  ExtrusionCrossSection=[1 1; -1 1; -1 -1; 1 -1]  ExtrusionCrossSectionUnits=m  ExtrusionLength=1  ExtrusionLengthUnits=m  PolygonNumSides=3  PolygonOuterRadius=1  PolygonOuterRadiusUnits=m  ExtGeomFileType=STL  ExtGeomFileName=geometry/Float.stl  ExtGeomFileUnits=m  RevolutionCrossSection=[1 1; 1 -1; 2 -1; 2 1]  RevolutionCrossSectionUnits=m  RevolutionExtent=Full  RevolutionAngle=180  RevolutionAngleUnits=deg
  External Force and Torque : sm_lib/Forces and Torques/External Force and Torque  ForceResolutionFrame=World  EnableForceX=off  EnableForceY=off  EnableForceZ=off  EnableForce=on  TorqueResolutionFrame=World  EnableTorqueX=off  EnableTorqueY=off  EnableTorqueZ=off  EnableTorque=on
  Motion Sensor : Subsystem
  Rigid Transform (Setup CG) : sm_lib/Frames and Transforms/Rigid Transform  TranslationMethod=Cartesian  TranslationStandardOffset=0  TranslationLengthUnit=m  TranslationStandardAxis=+Z  TranslationCartesianOffset=body.cg  TranslationROffset=0  TranslationROffsetUnits=m  TranslationZOffset=0  TranslationZOffsetUnits=m  TranslationThetaOffset=0  TranslationThetaOffsetUnits=deg  RotationMethod=None  RotationAngleUnits=rad  RotationStandardAxis=+Y  RotationAngle=0.05  RotationArbitraryAxis=[0.57735026918962584 0.57735026918962584 0.57735026918962584]  FollAlignAxisA=+X  BaseAlignAxisA=+Y  FollAlignAxisB=+Y  BaseAlignAxisB=+Z  RotationSequenceAxes=FollowerAxes  RotationSequence=XYX  RotationSequenceAngles=[0 0 0]  RotationSequenceAnglesUnits=deg  RotationMatrix=[1 0 0; 0 1 0; 0 0 1]
  Rigid Transform (Setup Initial Disp) : sm_lib/Frames and Transforms/Rigid Transform  TranslationMethod=Cartesian  TranslationStandardOffset=0  TranslationLengthUnit=m  TranslationStandardAxis=+Z  TranslationCartesianOffset=body.initDisp.initLinDisp  TranslationROffset=0  TranslationROffsetUnits=m  TranslationZOffset=0  TranslationZOffsetUnits=m  TranslationThetaOffset=0  TranslationThetaOffsetUnits=deg  RotationMethod=ArbitraryAxis  RotationAngleUnits=rad  RotationStandardAxis=+Y  RotationAngle=body.initDisp.initAngularDispAngle  RotationArbitraryAxis=body.initDisp.initAngularDispAxis  FollAlignAxisA=+X  BaseAlignAxisA=+Y  FollAlignAxisB=+Y  BaseAlignAxisB=+Z  RotationSequenceAxes=FollowerAxes  RotationSequence=XYX  RotationSequenceAngles=[0 0 0]  RotationSequenceAnglesUnits=deg  RotationMatrix=[1 0 0; 0 1 0; 0 0 1]
  Selector : Selector  InputPortWidth=6  IndexOptions=Index vector (dialog)  Indices=[1:3]  OutputSizes=1
  Selector1 : Selector  InputPortWidth=6  IndexOptions=Index vector (dialog)  Indices=[4:6]  OutputSizes=1
  Simulink-PS Converter1 : nesl_utility/Simulink-PS Converter  PhysicalDomain=network_engine_domain  SubClassName=ps_input  LeftPortType=input  RightPortType=output  PseudoPeriodic=off  Frequencies=[]  NoiseDistribution=none  NoiseParameters=[]  Unit=1  AffineConversion=off  FilteringAndDerivatives=zero  SimscapeFilterOrder=1  InputFilterTimeConstant=0.001  UdotUserProvided=1
  Simulink-PS Converter2 : nesl_utility/Simulink-PS Converter  PhysicalDomain=network_engine_domain  SubClassName=ps_input  LeftPortType=input  RightPortType=output  PseudoPeriodic=off  Frequencies=[]  NoiseDistribution=none  NoiseParameters=[]  Unit=1  AffineConversion=off  FilteringAndDerivatives=zero  SimscapeFilterOrder=1  InputFilterTimeConstant=0.001  UdotUserProvided=1
  World Frame : sm_lib/Frames and Transforms/World Frame
  Conn Free Surface : PMIOPort  Side=Right
  Response : Outport
  wires:
  Total Force/1 -> Selector1/1, Selector/1
  Selector/1 -> Simulink-PS Converter1/1
  Selector1/1 -> Simulink-PS Converter2/1
  Motion Sensor/1(Response) -> Response/1
  connections:
  External Force and Torque/LConn1 -- Simulink-PS Converter1/RConn1
  External Force and Torque/LConn2 -- Simulink-PS Converter2/RConn1
  Rigid Transform (Setup Initial Disp)/RConn1 -- Body Properties/RConn1 -- External Force and Torque/RConn1 -- Motion Sensor/RConn1
  Conn Free Surface/RConn1 -- Rigid Transform (Setup CG)/LConn1
  Rigid Transform (Setup Initial Disp)/LConn1 -- Rigid Transform (Setup CG)/RConn1
  World Frame/RConn1 -- Motion Sensor/LConn1

== system WaveStar/Float/Hydrodynamic Body/Wave Diffraction and Excitation Force Calculation ==
  Time : Inport
  Displacement : Inport  Port=2
  WaveElv : Inport  Port=3
  Add : Sum
  If2 : If  NumInputs=2  IfExpression=u1 < u2
  Linear Wave Excitation Force Variant Subsystem : Subsystem  Variant=on
  Merge1 : Merge
  No Ramp Function : Subsystem  TreatAsAtomicUnit=on
  Nonlinear FK Force Variant Subsystem : Subsystem  Variant=on
  Product : Product
  Ramp Function : Subsystem  TreatAsAtomicUnit=on
  Ramp Function Time : Constant  Value=simu.rampTime
  F_Excitation : Outport  PortDimensions=body.dof
  wires:
  Nonlinear FK Force Variant Subsystem/1(Nonlinear Excitation) -> Add/2
  Linear Wave Excitation Force Variant Subsystem/1(Linear Excitation) -> Add/1
  WaveElv/1 -> Nonlinear FK Force Variant Subsystem/3(WaveElv)
  Displacement/1 -> Nonlinear FK Force Variant Subsystem/2(Displacement)
  Product/1 -> F_Excitation/1  "F_Excitation"
  Add/1 -> Product/2  "F_wave"
  Time/1 -> If2/1, Ramp Function/1(Time), Nonlinear FK Force Variant Subsystem/1(Time), Linear Wave Excitation Force Variant Subsystem/1(Time)
  Merge1/1 -> Product/1  "R"
  Ramp Function Time/1 -> If2/2
  If2/2 -> No Ramp Function/Action
  If2/1 -> Ramp Function/Action
  Ramp Function/1(R) -> Merge1/1
  No Ramp Function/1(R) -> Merge1/2

== system WaveStar/Float/Hydrodynamic Body/Wave Radiation Forces Calculation ==
  Velocity : Inport
  Acceleration : Inport  Port=2
  Time : Inport  Port=3
  Added Mass Matrix : Constant  Value=body.hydroForce.fAddedMass
  Product1 : Product  Multiplication=Matrix(*)
  SS CI and Constant-Damping-CoeVariant Subsystem : Subsystem  Variant=on
  Transport Delay : TransportDelay  DelayTime=10e-8
  F_RadiationDamping : Outport
  F_AddedMass : Outport  Port=2
  wires:
  Time/1 -> SS CI and Constant-Damping-CoeVariant Subsystem/2(In2)
  Acceleration/1 -> Transport Delay/1
  Transport Delay/1 -> Product1/2
  SS CI and Constant-Damping-CoeVariant Subsystem/1(Out1) -> F_RadiationDamping/1  "F_RadiationDamping"
  Velocity/1 -> SS CI and Constant-Damping-CoeVariant Subsystem/1(In1)
  Product1/1 -> F_AddedMass/1  "F_AddedMass"
  Added Mass Matrix/1 -> Product1/1
